simulink model "XBATT07_reference_harness"  (R2025a)
settings: Solver=FixedStepDiscrete  StartTime=0.0  StopTime=25  FixedStep=0.1  RelTol=1e-3
undefined symbols (not defined in the file): SRE
settings Model: DataDictionary=Shared_DD.sldd  Creator=SimuVerity Contributors  LastModifiedBy=SimuVerity Contributors

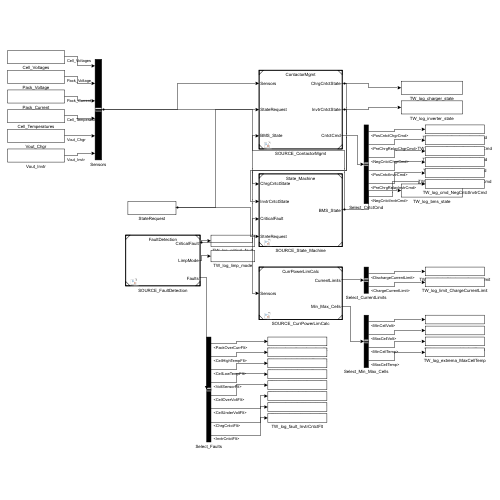
[thumbnail: Simulink's stored preview of the top-level diagram]
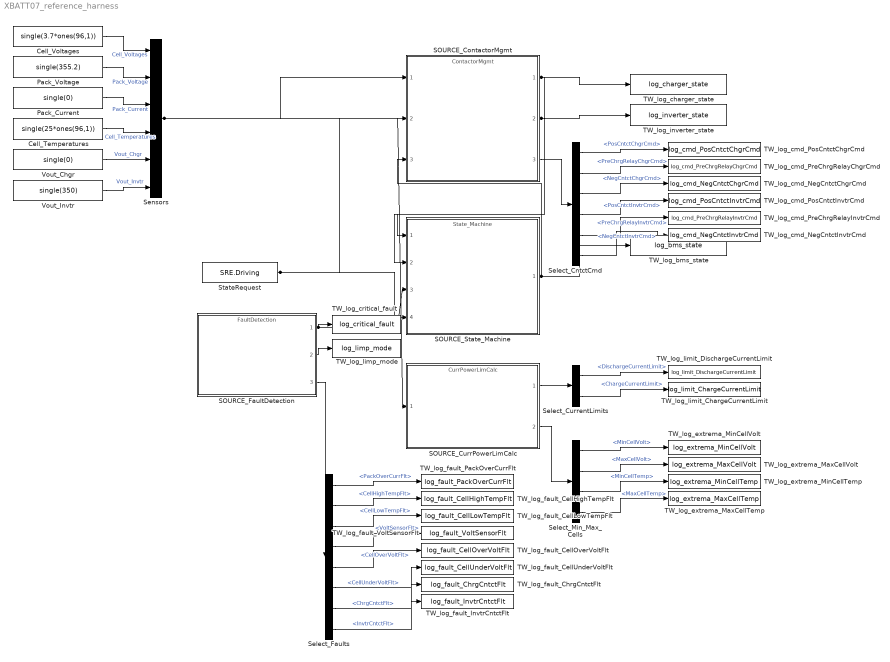
== system XBATT07_reference_harness ==
  Cell_Temperatures : Constant  Value=single(25*ones(96,1))
  Cell_Voltages : Constant  Value=single(3.7*ones(96,1))
  Pack_Current : Constant  Value=single(0)
  Pack_Voltage : Constant  Value=single(355.2)
  SOURCE_ContactorMgmt : ModelReference  ModelNameDialog=ContactorMgmt  SimulationMode=Normal  ModelReferenceVersion=5.15
  SOURCE_CurrPowerLimCalc : ModelReference  ModelNameDialog=CurrPowerLimCalc  SimulationMode=Normal  ModelReferenceVersion=5.31
  SOURCE_FaultDetection : ModelReference  ModelNameDialog=FaultDetection  SimulationMode=Normal  ModelReferenceVersion=5.25
  SOURCE_State_Machine : ModelReference  ModelNameDialog=State_Machine  SimulationMode=Normal  ModelReferenceVersion=5.3
  Select_CntctCmd : BusSelector  OutputSignals=PosCntctChgrCmd,PreChrgRelayChgrCmd,NegCntctChgrCmd,PosCntctInvtrCmd,PreChrgRelayInvtrCmd,NegCntctInvtrCmd
  Select_CurrentLimits : BusSelector  OutputSignals=DischargeCurrentLimit,ChargeCurrentLimit
  Select_Faults : BusSelector  OutputSignals=PackOverCurrFlt,CellHighTempFlt,CellLowTempFlt,VoltSensorFlt,CellOverVoltFlt,CellUnderVoltFlt,ChrgCntctFlt,InvtrCntctFlt
  Select_Min_Max_Cells : BusSelector  OutputSignals=MinCellVolt,MaxCellVolt,MinCellTemp,MaxCellTemp
  Sensors : BusCreator  Inputs=6  OutDataTypeStr=Bus: Sensors  NonVirtualBus=on
  StateRequest : Constant  Value=SRE.Driving  OutDataTypeStr=Enum: SRE
  TW_log_bms_state : ToWorkspace  VariableName=log_bms_state  SaveFormat=Timeseries  SampleTime=-1
  TW_log_charger_state : ToWorkspace  VariableName=log_charger_state  SaveFormat=Timeseries  SampleTime=-1
  TW_log_cmd_NegCntctChgrCmd : ToWorkspace  VariableName=log_cmd_NegCntctChgrCmd  SaveFormat=Timeseries  SampleTime=-1
  TW_log_cmd_NegCntctInvtrCmd : ToWorkspace  VariableName=log_cmd_NegCntctInvtrCmd  SaveFormat=Timeseries  SampleTime=-1
  TW_log_cmd_PosCntctChgrCmd : ToWorkspace  VariableName=log_cmd_PosCntctChgrCmd  SaveFormat=Timeseries  SampleTime=-1
  TW_log_cmd_PosCntctInvtrCmd : ToWorkspace  VariableName=log_cmd_PosCntctInvtrCmd  SaveFormat=Timeseries  SampleTime=-1
  TW_log_cmd_PreChrgRelayChgrCmd : ToWorkspace  VariableName=log_cmd_PreChrgRelayChgrCmd  SaveFormat=Timeseries  SampleTime=-1
  TW_log_cmd_PreChrgRelayInvtrCmd : ToWorkspace  VariableName=log_cmd_PreChrgRelayInvtrCmd  SaveFormat=Timeseries  SampleTime=-1
  TW_log_critical_fault : ToWorkspace  VariableName=log_critical_fault  SaveFormat=Timeseries  SampleTime=-1
  TW_log_extrema_MaxCellTemp : ToWorkspace  VariableName=log_extrema_MaxCellTemp  SaveFormat=Timeseries  SampleTime=-1
  TW_log_extrema_MaxCellVolt : ToWorkspace  VariableName=log_extrema_MaxCellVolt  SaveFormat=Timeseries  SampleTime=-1
  TW_log_extrema_MinCellTemp : ToWorkspace  VariableName=log_extrema_MinCellTemp  SaveFormat=Timeseries  SampleTime=-1
  TW_log_extrema_MinCellVolt : ToWorkspace  VariableName=log_extrema_MinCellVolt  SaveFormat=Timeseries  SampleTime=-1
  TW_log_fault_CellHighTempFlt : ToWorkspace  VariableName=log_fault_CellHighTempFlt  SaveFormat=Timeseries  SampleTime=-1
  TW_log_fault_CellLowTempFlt : ToWorkspace  VariableName=log_fault_CellLowTempFlt  SaveFormat=Timeseries  SampleTime=-1
  TW_log_fault_CellOverVoltFlt : ToWorkspace  VariableName=log_fault_CellOverVoltFlt  SaveFormat=Timeseries  SampleTime=-1
  TW_log_fault_CellUnderVoltFlt : ToWorkspace  VariableName=log_fault_CellUnderVoltFlt  SaveFormat=Timeseries  SampleTime=-1
  TW_log_fault_ChrgCntctFlt : ToWorkspace  VariableName=log_fault_ChrgCntctFlt  SaveFormat=Timeseries  SampleTime=-1
  TW_log_fault_InvtrCntctFlt : ToWorkspace  VariableName=log_fault_InvtrCntctFlt  SaveFormat=Timeseries  SampleTime=-1
  TW_log_fault_PackOverCurrFlt : ToWorkspace  VariableName=log_fault_PackOverCurrFlt  SaveFormat=Timeseries  SampleTime=-1
  TW_log_fault_VoltSensorFlt : ToWorkspace  VariableName=log_fault_VoltSensorFlt  SaveFormat=Timeseries  SampleTime=-1
  TW_log_inverter_state : ToWorkspace  VariableName=log_inverter_state  SaveFormat=Timeseries  SampleTime=-1
  TW_log_limit_ChargeCurrentLimit : ToWorkspace  VariableName=log_limit_ChargeCurrentLimit  SaveFormat=Timeseries  SampleTime=-1
  TW_log_limit_DischargeCurrentLimit : ToWorkspace  VariableName=log_limit_DischargeCurrentLimit  SaveFormat=Timeseries  SampleTime=-1
  TW_log_limp_mode : ToWorkspace  VariableName=log_limp_mode  SaveFormat=Timeseries  SampleTime=-1
  Vout_Chgr : Constant  Value=single(0)
  Vout_Invtr : Constant  Value=single(350)
  wires:
  Cell_Voltages/1 -> Sensors/1  "Cell_Voltages"
  Pack_Voltage/1 -> Sensors/2  "Pack_Voltage"
  Pack_Current/1 -> Sensors/3  "Pack_Current"
  Cell_Temperatures/1 -> Sensors/4  "Cell_Temperatures"
  Vout_Chgr/1 -> Sensors/5  "Vout_Chgr"
  Vout_Invtr/1 -> Sensors/6  "Vout_Invtr"
  Sensors/1 -> SOURCE_ContactorMgmt/1, SOURCE_CurrPowerLimCalc/1
  SOURCE_ContactorMgmt/1 -> SOURCE_State_Machine/1, TW_log_charger_state/1
  SOURCE_ContactorMgmt/2 -> SOURCE_State_Machine/2, TW_log_inverter_state/1
  SOURCE_FaultDetection/1 -> SOURCE_State_Machine/3, TW_log_critical_fault/1
  StateRequest/1 -> SOURCE_State_Machine/4, SOURCE_ContactorMgmt/2
  SOURCE_State_Machine/1 -> SOURCE_ContactorMgmt/3, TW_log_bms_state/1
  SOURCE_ContactorMgmt/3 -> Select_CntctCmd/1
  Select_CntctCmd/1 -> TW_log_cmd_PosCntctChgrCmd/1  "<PosCntctChgrCmd>"
  Select_CntctCmd/2 -> TW_log_cmd_PreChrgRelayChgrCmd/1  "<PreChrgRelayChgrCmd>"
  Select_CntctCmd/3 -> TW_log_cmd_NegCntctChgrCmd/1  "<NegCntctChgrCmd>"
  Select_CntctCmd/4 -> TW_log_cmd_PosCntctInvtrCmd/1  "<PosCntctInvtrCmd>"
  Select_CntctCmd/5 -> TW_log_cmd_PreChrgRelayInvtrCmd/1  "<PreChrgRelayInvtrCmd>"
  Select_CntctCmd/6 -> TW_log_cmd_NegCntctInvtrCmd/1  "<NegCntctInvtrCmd>"
  SOURCE_CurrPowerLimCalc/1 -> Select_CurrentLimits/1
  Select_CurrentLimits/1 -> TW_log_limit_DischargeCurrentLimit/1  "<DischargeCurrentLimit>"
  Select_CurrentLimits/2 -> TW_log_limit_ChargeCurrentLimit/1  "<ChargeCurrentLimit>"
  SOURCE_CurrPowerLimCalc/2 -> Select_Min_Max_Cells/1
  Select_Min_Max_Cells/1 -> TW_log_extrema_MinCellVolt/1  "<MinCellVolt>"
  Select_Min_Max_Cells/2 -> TW_log_extrema_MaxCellVolt/1  "<MaxCellVolt>"
  Select_Min_Max_Cells/3 -> TW_log_extrema_MinCellTemp/1  "<MinCellTemp>"
  Select_Min_Max_Cells/4 -> TW_log_extrema_MaxCellTemp/1  "<MaxCellTemp>"
  SOURCE_FaultDetection/2 -> TW_log_limp_mode/1
  SOURCE_FaultDetection/3 -> Select_Faults/1
  Select_Faults/1 -> TW_log_fault_PackOverCurrFlt/1  "<PackOverCurrFlt>"
  Select_Faults/2 -> TW_log_fault_CellHighTempFlt/1  "<CellHighTempFlt>"
  Select_Faults/3 -> TW_log_fault_CellLowTempFlt/1  "<CellLowTempFlt>"
  Select_Faults/4 -> TW_log_fault_VoltSensorFlt/1  "<VoltSensorFlt>"
  Select_Faults/5 -> TW_log_fault_CellOverVoltFlt/1  "<CellOverVoltFlt>"
  Select_Faults/6 -> TW_log_fault_CellUnderVoltFlt/1  "<CellUnderVoltFlt>"
  Select_Faults/7 -> TW_log_fault_ChrgCntctFlt/1  "<ChrgCntctFlt>"
  Select_Faults/8 -> TW_log_fault_InvtrCntctFlt/1  "<InvtrCntctFlt>"
